simulink model "buck_circuito_completo"  (R2026a)
settings: Solver=ode23t  StopTime=12e-3  MaxStep=1e-6  RelTol=1e-4
PreLoadFcn:
  | circuito_completo_parametros;
values from neighbouring files (symbols this model uses):
  ADC_A_UV = 389000    [circuito_completo_parametros.m]
  ADC_B_X1E5 = 8251    [circuito_completo_parametros.m]
  D_FIXO_PERMIL = 500    [circuito_completo_parametros.m]
  MODO = 1    [circuito_completo.m]    (also in circuito_completo_parametros.m = 0)
  R_pot = 46.6    [circuito_completo_parametros.m]
  T_KEY = 0    [circuito_completo.m]    (also in circuito_completo_parametros.m = 0.001)
  Ts = 1e-4    (= 0.0001)    [circuito_completo_parametros.m]    (also in etapa01_referencia.m; etapa02_projeto_buck.m; etapa02_simulink.m; etapa03_projeto_ccs.m)
libraries: fl_lib x69, nesl_utility x15, ee_lib x10, simulink x1
(part 1 of 2)
settings Model: Creator=pedro  LastModifiedBy=pedro

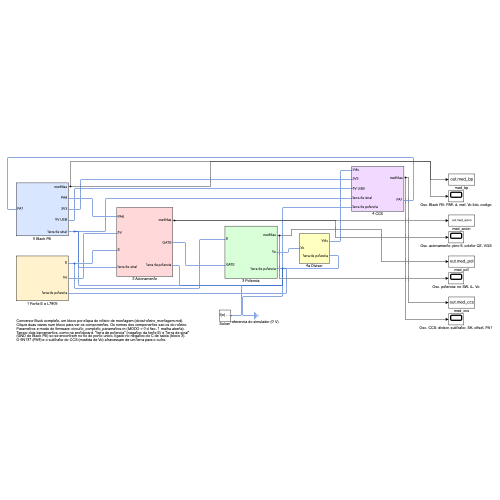
[thumbnail: Simulink's stored preview of the top-level diagram]
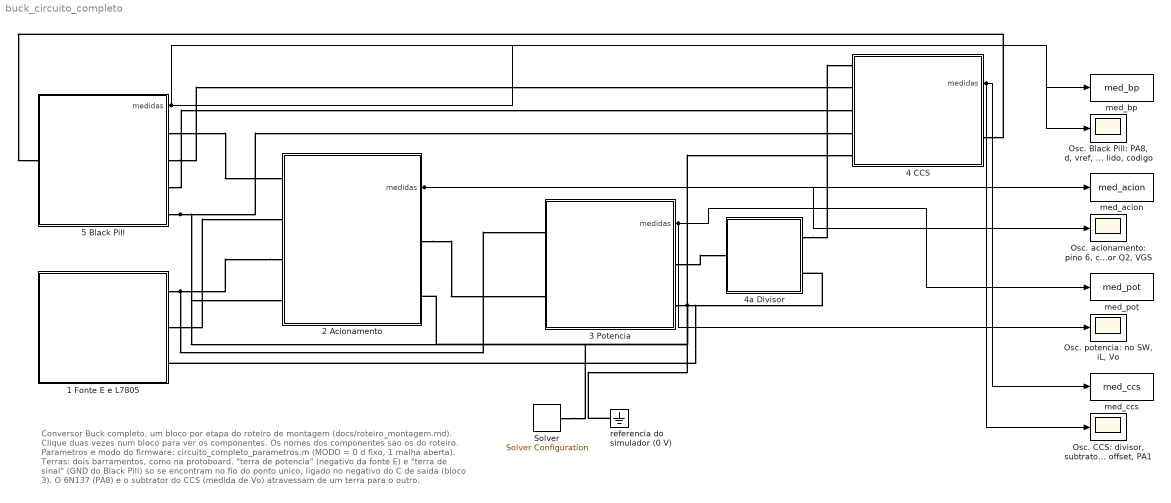
== system buck_circuito_completo ==
  note: Conversor Buck completo, um bloco por etapa do roteiro de montagem (docs/roteiro_montagem.md).
      | Clique duas vezes num bloco para ver os componentes. Os nomes dos componentes sao os do roteiro.
      | Parametros e modo do firmware: circuito_completo_parametros.m (MODO = 0 d fixo, 1 malha aberta).
      | Terras: dois barramentos, como na protoboard. "terra de potencia" (negativo da fonte E) e "terra de sinal"
      | (GND do Black Pill) so se encontram no fio do ponto unico, ligado no negativo do C de saida (bloco 3).
      | O 6N137 (PA8) e o subtrator do CCS (medida de Vo) atravessam de um terra para o outro.
  1 Fonte E e L7805 : Subsystem
  2 Acionamento : Subsystem
  3 Potencia : Subsystem
  4 CCS : Subsystem
  4a Divisor : Subsystem
  5 Black Pill : Subsystem
  "Osc. Black Pill: PA8, d, vref, Vo lido, codigo" : Scope
  "Osc. CCS: divisor, subtrator, SK, offset, PA1" : Scope
  "Osc. acionamento: pino 6, coletor Q2, VGS" : Scope
  "Osc. potencia: no SW, iL, Vo" : Scope
  Solver : nesl_utility/Solver Configuration  PhysicalDomain=network_engine_domain  SubClassName=solver  LeftPortType=input  RightPortType=generic  Tones=[]  Harmonics=[]  SimulateNoise=off  Profile=off  UseLocalSampling=off  EnableSwitchedLinearOptims=on  FrequencyDomain=off  UseCCode=off  RelTol=0.001  AbsTol=0.001  MinStep=1e-09  ToWorkspace=off  RevertToSquareIcSolve=off  NumHomotopyIterations=100  PhasorMode=off  PhasorModeNumHarmonics=1  ConsistencySolver=NEWTON_XTOL_AFTER_FTOL  CanonicalOrdering=CANONICAL  OptimizeIntermediates=OPTIMIZED  IndexReductionMethod=DerivativeReplacement  DoDC=off  ResidualTolerance=1e-09  ConsistencyTolSource=GLOBAL  ConsistencyAbsTol=0.001  ConsistencyRelTol=0.001  ConsistencyTolFactor=0.001  UseLocalSolver=off  LocalSolverChoice=NE_BACKWARD_EULER_ADVANCER  ResolveIndetEquations=on  FunctionEvalNumThread=1  LocalSolverSampleTime=0.001  DoFixedCost=off  MaxNonlinIter=3  MaxModeIter=2  ComputeImpulses=off  ImpulseIterations=2  LinearAlgebra=auto  LinearAlgebraNumThread=0  EquationFormulation=NE_TIME_EF  DelaysMemoryBudget=1024  AutomaticFiltering=on  FilteringTimeConstant=0.001  PartitionStorageMethod=AS_NEEDED  PartitionMemoryBudget=1024  PartitionMethod=ROBUST  MultibodyUseLocalSolver=off  MultibodyLocalSolverChoice=ODE1  MultibodyLocalSolverSampleTime=0.001
  med_acion : ToWorkspace  VariableName=med_acion  SaveFormat=Timeseries  SampleTime=-1
  med_bp : ToWorkspace  VariableName=med_bp  SaveFormat=Timeseries  SampleTime=-1
  med_ccs : ToWorkspace  VariableName=med_ccs  SaveFormat=Timeseries  SampleTime=-1
  med_pot : ToWorkspace  VariableName=med_pot  SaveFormat=Timeseries  SampleTime=-1
  referencia do simulador (0 V) : fl_lib/Electrical/Electrical Elements/Electrical Reference
  wires:
  5 Black Pill/1(medidas) -> med_bp/1, "Osc. Black Pill: PA8, d, vref, Vo lido, codigo"/1
  2 Acionamento/1(medidas) -> med_acion/1, "Osc. acionamento: pino 6, coletor Q2, VGS"/1
  3 Potencia/1(medidas) -> med_pot/1, "Osc. potencia: no SW, iL, Vo"/1
  4 CCS/1(medidas) -> med_ccs/1, "Osc. CCS: divisor, subtrator, SK, offset, PA1"/1
  connections:
  2 Acionamento/LConn3 -- 1 Fonte E e L7805/RConn1 -- 3 Potencia/LConn1
  1 Fonte E e L7805/RConn2 -- 2 Acionamento/LConn2
  5 Black Pill/RConn1 -- 2 Acionamento/LConn1
  2 Acionamento/RConn1 -- 3 Potencia/LConn2
  3 Potencia/RConn1 -- 4a Divisor/LConn1
  4a Divisor/RConn1 -- 4 CCS/LConn1
  5 Black Pill/RConn2 -- 4 CCS/LConn2
  5 Black Pill/RConn3 -- 4 CCS/LConn3
  4 CCS/RConn1 -- 5 Black Pill/LConn1
  1 Fonte E e L7805/RConn3 -- 3 Potencia/RConn2 -- 2 Acionamento/RConn2 -- 4a Divisor/RConn2 -- 4 CCS/LConn5 -- 5 Black Pill/RConn4 -- 2 Acionamento/LConn4 -- 4 CCS/LConn4 -- referencia do simulador (0 V)/LConn1 -- Solver/RConn1

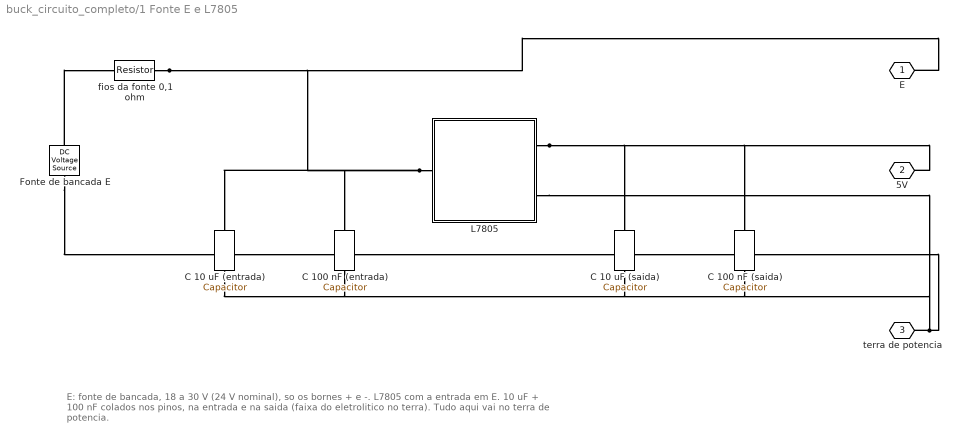
== system buck_circuito_completo/1 Fonte E e L7805 ==
  note: E: fonte de bancada, 18 a 30 V (24 V nominal), so os bornes + e -.
      | L7805 com a entrada em E. 10 uF + 100 nF colados nos pinos, na entrada e na saida (faixa do eletrolitico no terra).
      | Tudo aqui vai no terra de potencia.
  C 10 uF (entrada) : fl_lib/Electrical/Electrical Elements/Capacitor  c=10e-6 F  r=0.3 Ohm  g=0 1/Ohm  i_specify=off  i_priority=None  i=0 A  i_nominal_specify=off  i_nominal_value=1  i_nominal_unit=A  v_specify=off  v_priority=None  v=0 V  v_nominal_specify=off  v_nominal_value=1  v_nominal_unit=V  vc_specify=off  vc_priority=High  vc=0 V  vc_nominal_specify=off  vc_nominal_value=1  vc_nominal_unit=V
  C 10 uF (saida) : fl_lib/Electrical/Electrical Elements/Capacitor  c=10e-6 F  r=0.3 Ohm  g=0 1/Ohm  i_specify=off  i_priority=None  i=0 A  i_nominal_specify=off  i_nominal_value=1  i_nominal_unit=A  v_specify=off  v_priority=None  v=0 V  v_nominal_specify=off  v_nominal_value=1  v_nominal_unit=V  vc_specify=off  vc_priority=High  vc=0 V  vc_nominal_specify=off  vc_nominal_value=1  vc_nominal_unit=V
  C 100 nF (entrada) : fl_lib/Electrical/Electrical Elements/Capacitor  c=100e-9 F  r=1e-6 Ohm  g=0 1/Ohm  i_specify=off  i_priority=None  i=0 A  i_nominal_specify=off  i_nominal_value=1  i_nominal_unit=A  v_specify=off  v_priority=None  v=0 V  v_nominal_specify=off  v_nominal_value=1  v_nominal_unit=V  vc_specify=off  vc_priority=High  vc=0 V  vc_nominal_specify=off  vc_nominal_value=1  vc_nominal_unit=V
  C 100 nF (saida) : fl_lib/Electrical/Electrical Elements/Capacitor  c=100e-9 F  r=1e-6 Ohm  g=0 1/Ohm  i_specify=off  i_priority=None  i=0 A  i_nominal_specify=off  i_nominal_value=1  i_nominal_unit=A  v_specify=off  v_priority=None  v=0 V  v_nominal_specify=off  v_nominal_value=1  v_nominal_unit=V  vc_specify=off  vc_priority=High  vc=0 V  vc_nominal_specify=off  vc_nominal_value=1  vc_nominal_unit=V
  Fonte de bancada E : fl_lib/Electrical/Electrical Sources/DC Voltage Source  v0=E V
  L7805 : Subsystem
  fios da fonte 0,1 ohm : fl_lib/Electrical/Electrical Elements/Resistor  R=0.1 Ohm  i_specify=off  i_priority=None  i=0 A  i_nominal_specify=off  i_nominal_value=1  i_nominal_unit=A  v_specify=off  v_priority=None  v=0 V  v_nominal_specify=off  v_nominal_value=1  v_nominal_unit=V
  E : PMIOPort  Side=Right
  5V : PMIOPort  Port=2  Side=Right
  terra de potencia : PMIOPort  Port=3  Side=Right
  connections:
  Fonte de bancada E/LConn1 -- fios da fonte 0,1 ohm/LConn1
  E/RConn1 -- fios da fonte 0,1 ohm/RConn1 -- C 10 uF (entrada)/LConn1 -- L7805/LConn1 -- C 100 nF (entrada)/LConn1
  Fonte de bancada E/RConn1 -- L7805/RConn2 -- C 10 uF (entrada)/RConn1 -- C 100 nF (entrada)/RConn1 -- C 10 uF (saida)/RConn1 -- terra de potencia/RConn1 -- C 100 nF (saida)/RConn1
  5V/RConn1 -- L7805/RConn1 -- C 10 uF (saida)/LConn1 -- C 100 nF (saida)/LConn1

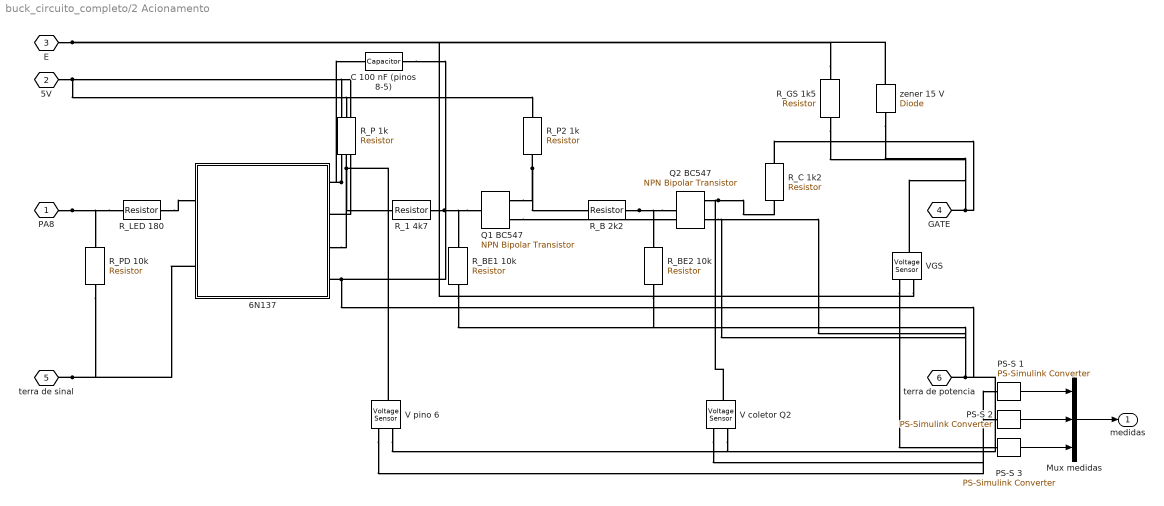
== system buck_circuito_completo/2 Acionamento ==
  6N137 : Subsystem
  C 100 nF (pinos 8-5) : fl_lib/Electrical/Electrical Elements/Capacitor  c=100e-9 F  r=1e-6 Ohm  g=0 1/Ohm  i_specify=off  i_priority=None  i=0 A  i_nominal_specify=off  i_nominal_value=1  i_nominal_unit=A  v_specify=off  v_priority=None  v=0 V  v_nominal_specify=off  v_nominal_value=1  v_nominal_unit=V  vc_specify=off  vc_priority=High  vc=0 V  vc_nominal_specify=off  vc_nominal_value=1  vc_nominal_unit=V
  Mux medidas : Mux  Inputs=3
  PS-S 1 : nesl_utility/PS-Simulink Converter  PhysicalDomain=network_engine_domain  SubClassName=ps_output  LeftPortType=input  RightPortType=output  PseudoPeriodic=off  Frequencies=[]  VectorFormat=inherit  Unit=V  AffineConversion=off
  PS-S 2 : nesl_utility/PS-Simulink Converter  PhysicalDomain=network_engine_domain  SubClassName=ps_output  LeftPortType=input  RightPortType=output  PseudoPeriodic=off  Frequencies=[]  VectorFormat=inherit  Unit=V  AffineConversion=off
  PS-S 3 : nesl_utility/PS-Simulink Converter  PhysicalDomain=network_engine_domain  SubClassName=ps_output  LeftPortType=input  RightPortType=output  PseudoPeriodic=off  Frequencies=[]  VectorFormat=inherit  Unit=V  AffineConversion=off
  Q1 BC547 : ee_lib/Semiconductors & Converters/NPN Bipolar Transistor  parameterization=1  BF=100  IS=1e-14 A  VAF=200 V  hfe=100  hoe=50e-6 1/Ohm  Ic_h=1 mA  Vce_h=5 V  V1=0.55 V  I1=0.5 mA  BR=1  Tmeas=25 degC  RC=0.01 Ohm  RE=1e-4 Ohm  RB=1 Ohm  C_BC=5 pF  C_BE=5 pF  TF=0 us  TR=0 us  prmDatasheet=1  prmEquCoeff=1  hfe_T2=125  XTB=0  V1_T2=0.45 V  I1_T2=0.5 mA  Tmeas2=125 degC  EG=1.11 eV  XTI=3  TdeviceDatasheet=25 degC  TdeviceEquCoeff=25 degC  ec=1  ib_specify=off  ib_priority=None  ib=0 A  ib_nominal_specify=off  ib_nominal_value=1  ib_nominal_unit=A  ic_specify=off  ic_priority=None  ic=0 A  ic_nominal_specify=off  ic_nominal_value=1  ic_nominal_unit=A  vce_specify=off  vce_priority=None  vce=0 V  vce_nominal_specify=off  vce_nominal_value=1  vce_nominal_unit=V  vbe_specify=off  vbe_priority=None  vbe=0 V  vbe_nominal_specify=off  vbe_nominal_value=1  vbe_nominal_unit=V  Qbc_specify=off  Qbc_priority=High  Qbc=0 C  Qbc_nominal_specify=off  Qbc_nominal_value=1  Qbc_nominal_unit=uC  Qbe_specify=off  Qbe_priority=High  Qbe=0 C  Qbe_nominal_specify=off  Qbe_nominal_value=1  Qbe_nominal_unit=uC  thermal_network_parameterization=ee.enum.thermalNetworkTopology.junctionCase  Rth=[0, 10] K/W  Rth_Cauer=[1, 3, 10] K/W  Rth_Foster=[.08, .14, .22, .16] K/W  thermal_mass_parameterization=ee.enum.thermalNetwork.timeconstant  thermal_mass=[0, 1] J/K  thermal_mass_Cauer=[.1, .3, 1] J/K  thermal_mass_Foster=[.001, .005, .05, .5] J/K  thermal_time_constant=[0, 10] s  thermal_time_constant_Cauer=[1, 3, 10] s  thermal_time_constant_Foster=[7e-05, .0007, .01, .08] s  thermal_mass_initial_temperatures=[25, 25] degC  thermal_mass_initial_temperatures_Cauer=[25, 25, 25] degC  Tvec_initial_Foster=[25, 25, 25, 25] degC
  Q2 BC547 : ee_lib/Semiconductors & Converters/NPN Bipolar Transistor  parameterization=1  BF=100  IS=1e-14 A  VAF=200 V  hfe=100  hoe=50e-6 1/Ohm  Ic_h=1 mA  Vce_h=5 V  V1=0.55 V  I1=0.5 mA  BR=1  Tmeas=25 degC  RC=0.01 Ohm  RE=1e-4 Ohm  RB=1 Ohm  C_BC=5 pF  C_BE=5 pF  TF=0 us  TR=0 us  prmDatasheet=1  prmEquCoeff=1  hfe_T2=125  XTB=0  V1_T2=0.45 V  I1_T2=0.5 mA  Tmeas2=125 degC  EG=1.11 eV  XTI=3  TdeviceDatasheet=25 degC  TdeviceEquCoeff=25 degC  ec=1  ib_specify=off  ib_priority=None  ib=0 A  ib_nominal_specify=off  ib_nominal_value=1  ib_nominal_unit=A  ic_specify=off  ic_priority=None  ic=0 A  ic_nominal_specify=off  ic_nominal_value=1  ic_nominal_unit=A  vce_specify=off  vce_priority=None  vce=0 V  vce_nominal_specify=off  vce_nominal_value=1  vce_nominal_unit=V  vbe_specify=off  vbe_priority=None  vbe=0 V  vbe_nominal_specify=off  vbe_nominal_value=1  vbe_nominal_unit=V  Qbc_specify=off  Qbc_priority=High  Qbc=0 C  Qbc_nominal_specify=off  Qbc_nominal_value=1  Qbc_nominal_unit=uC  Qbe_specify=off  Qbe_priority=High  Qbe=0 C  Qbe_nominal_specify=off  Qbe_nominal_value=1  Qbe_nominal_unit=uC  thermal_network_parameterization=ee.enum.thermalNetworkTopology.junctionCase  Rth=[0, 10] K/W  Rth_Cauer=[1, 3, 10] K/W  Rth_Foster=[.08, .14, .22, .16] K/W  thermal_mass_parameterization=ee.enum.thermalNetwork.timeconstant  thermal_mass=[0, 1] J/K  thermal_mass_Cauer=[.1, .3, 1] J/K  thermal_mass_Foster=[.001, .005, .05, .5] J/K  thermal_time_constant=[0, 10] s  thermal_time_constant_Cauer=[1, 3, 10] s  thermal_time_constant_Foster=[7e-05, .0007, .01, .08] s  thermal_mass_initial_temperatures=[25, 25] degC  thermal_mass_initial_temperatures_Cauer=[25, 25, 25] degC  Tvec_initial_Foster=[25, 25, 25, 25] degC
  R_1 4k7 : fl_lib/Electrical/Electrical Elements/Resistor  R=4.7e3 Ohm  i_specify=off  i_priority=None  i=0 A  i_nominal_specify=off  i_nominal_value=1  i_nominal_unit=A  v_specify=off  v_priority=None  v=0 V  v_nominal_specify=off  v_nominal_value=1  v_nominal_unit=V
  R_B 2k2 : fl_lib/Electrical/Electrical Elements/Resistor  R=2.2e3 Ohm  i_specify=off  i_priority=None  i=0 A  i_nominal_specify=off  i_nominal_value=1  i_nominal_unit=A  v_specify=off  v_priority=None  v=0 V  v_nominal_specify=off  v_nominal_value=1  v_nominal_unit=V
  R_BE1 10k : fl_lib/Electrical/Electrical Elements/Resistor  R=10e3 Ohm  i_specify=off  i_priority=None  i=0 A  i_nominal_specify=off  i_nominal_value=1  i_nominal_unit=A  v_specify=off  v_priority=None  v=0 V  v_nominal_specify=off  v_nominal_value=1  v_nominal_unit=V
  R_BE2 10k : fl_lib/Electrical/Electrical Elements/Resistor  R=10e3 Ohm  i_specify=off  i_priority=None  i=0 A  i_nominal_specify=off  i_nominal_value=1  i_nominal_unit=A  v_specify=off  v_priority=None  v=0 V  v_nominal_specify=off  v_nominal_value=1  v_nominal_unit=V
  R_C 1k2 : fl_lib/Electrical/Electrical Elements/Resistor  R=1.2e3 Ohm  i_specify=off  i_priority=None  i=0 A  i_nominal_specify=off  i_nominal_value=1  i_nominal_unit=A  v_specify=off  v_priority=None  v=0 V  v_nominal_specify=off  v_nominal_value=1  v_nominal_unit=V
  R_GS 1k5 : fl_lib/Electrical/Electrical Elements/Resistor  R=1.5e3 Ohm  i_specify=off  i_priority=None  i=0 A  i_nominal_specify=off  i_nominal_value=1  i_nominal_unit=A  v_specify=off  v_priority=None  v=0 V  v_nominal_specify=off  v_nominal_value=1  v_nominal_unit=V
  R_LED 180 : fl_lib/Electrical/Electrical Elements/Resistor  R=180 Ohm  i_specify=off  i_priority=None  i=0 A  i_nominal_specify=off  i_nominal_value=1  i_nominal_unit=A  v_specify=off  v_priority=None  v=0 V  v_nominal_specify=off  v_nominal_value=1  v_nominal_unit=V
  R_P 1k : fl_lib/Electrical/Electrical Elements/Resistor  R=1e3 Ohm  i_specify=off  i_priority=None  i=0 A  i_nominal_specify=off  i_nominal_value=1  i_nominal_unit=A  v_specify=off  v_priority=None  v=0 V  v_nominal_specify=off  v_nominal_value=1  v_nominal_unit=V
  R_P2 1k : fl_lib/Electrical/Electrical Elements/Resistor  R=1e3 Ohm  i_specify=off  i_priority=None  i=0 A  i_nominal_specify=off  i_nominal_value=1  i_nominal_unit=A  v_specify=off  v_priority=None  v=0 V  v_nominal_specify=off  v_nominal_value=1  v_nominal_unit=V
  R_PD 10k : fl_lib/Electrical/Electrical Elements/Resistor  R=10e3 Ohm  i_specify=off  i_priority=None  i=0 A  i_nominal_specify=off  i_nominal_value=1  i_nominal_unit=A  v_specify=off  v_priority=None  v=0 V  v_nominal_specify=off  v_nominal_value=1  v_nominal_unit=V
  V coletor Q2 : fl_lib/Electrical/Electrical Sensors/Voltage Sensor
  V pino 6 : fl_lib/Electrical/Electrical Sensors/Voltage Sensor
  VGS : fl_lib/Electrical/Electrical Sensors/Voltage Sensor
  zener 15 V : ee_lib/Semiconductors & Converters/Diode  ModelType=ee.enum.diode.modelType.pwl  TableType=ee.enum.diode.tableType.IfMat  IfMat=[.07, .12, .19, 1.75, 4.24, 7.32, 11.2; .16, .3, .72, 2.14, 5.02, 8.35, 13.12] A  VfMat=[.9, 1.15, 1.25, 1.5, 1.75, 2.17, 2.6, 2.85; .58, .68, .75, 1.1, 1.38, 1.77, 2.27, 2.7] V  TjVec=[25, 125] degC  VfVec=[.5, .7, .9, 1.3, 1.7, 2.1, 2.5] V  IfVec=[.1, .2, .5, 1, 2, 4, 7, 10] A  IrMat=[1e-06, 2e-06, 5e-06, 1e-05, 2.5e-05, 5e-05, .0001; 2e-06, 5e-06, 1e-05, 4e-05, 8e-05, .0002, .0005] A  VrMat=[10, 100, 200, 250, 300, 325, 350; 10, 70, 160, 220, 270, 300, 320] V  VrVec=[10, 20, 40, 50, 70, 80, 100] V  IrVec=[1e-06, 2e-06, 5e-06, 1e-05, 2e-05, 5e-05, .0001] A  Vf=0.7 V  Ron=0.5 Ohm  Goff=1e-8 S  prmExp=ee.enum.diode.expParam.useTwo  I12=[.0137, .545] A  V12=[.6, .7] V  RS=0 Ohm  Tmeas=298.15 K  IS=1e-12 A  ec=1  I1=0.0137 A  V1=0.6 V  N_series=1  N_parallel=1  ZenerEnable=true  Rz=1 Ohm  BV=15 V  C_param=ee.enum.diode.capParam.fixed  CJ=0 pF  CJ0=5 pF  Vvec=[.1, 10, 100] V  Cvec=[3.5, 1, .4] pF  VJ=1 V  Mgrad=0.5  FC=0.5  Q_param=ee.enum.diode.recoveryParam.off  iRM=-7.15 A  iF=4 A  didt=-750 A/us  trr_factor=3  trr=115 ns  Qrr=150 nA*s  Vr=-600 V  Ls=150 nH  Erec=0.03 J  TT=50 ns  tau=100 ns  T_param=ee.enum.diode.temperatureParam.off  Tdevice=298.15 K  I1_T2=0.245 A  V1_T2=0.5 V  IS_T2=1.25e-7 A  Tmeas2=125 degC  XTI_param=ee.enum.diode.xtiParam.pn  XTI=3  EG_param=ee.enum.diode.egapParam.material_si  EG=1.11 eV  dBVdT=0 V/K  enable_fault_input=simscape.enum.onoff.off  i_specify=off  i_priority=None  i=0 A  i_nominal_specify=off  i_nominal_value=1  i_nominal_unit=A  v_specify=off  v_priority=None  v=0 V  v_nominal_specify=off  v_nominal_value=1  v_nominal_unit=V  v_capacitor_specify=off  v_capacitor_priority=None  v_capacitor=0 V  v_capacitor_nominal_specify=off  v_capacitor_nominal_value=1  v_capacitor_nominal_unit=V  Qj_specify=off  Qj_priority=High  Qj=0 C  Qj_nominal_specify=off  Qj_nominal_value=1  Qj_nominal_unit=C  i_diode_specify=off  i_diode_priority=None  i_diode=0 A  i_diode_nominal_specify=off  i_diode_nominal_value=1  i_diode_nominal_unit=A  v_diode_specify=off  v_diode_priority=None  v_diode=0 V  v_diode_nominal_specify=off  v_diode_nominal_value=1  v_diode_nominal_unit=V  i_capacitor_specify=off  i_capacitor_priority=None  i_capacitor=0 A  i_capacitor_nominal_specify=off  i_capacitor_nominal_value=1  i_capacitor_nominal_unit=A  fidelity_level=ee.enum.diode.fidelity.includeChargeDyn  rec_loss_model=ee.enum.diode.reverseRecoveryModelTabulateUpTo3D.fixed  ErecVal=0 J  scaleWithIandV=true  ErecMat=zeros(2, 3) J  ErecMat3D=zeros(2, 3, 2) J  TjrecVec=[298.15, 398.15] K  IfrecVec=[.1, 1, 10] A  IrecVal=10 A  VrecVal=10 V  VrecVec=[0, 100] V  tFilter=1 / 1000 / 100 s  thermal_network_parameterization=ee.enum.thermalNetworkTopology.junctionCase  Rth=[0, 10] K/W  Rth_Cauer=[1, 3, 10] K/W  Rth_Foster=[.08, .14, .22, .16] K/W  thermal_mass_parameterization=ee.enum.thermalNetwork.timeconstant  thermal_mass=[0, 1] J/K  thermal_mass_Cauer=[.1, .3, 1] J/K  thermal_mass_Foster=[.001, .005, .05, .5] J/K  thermal_time_constant=[0, 10] s  thermal_time_constant_Cauer=[1, 3, 10] s  thermal_time_constant_Foster=[7e-05, .0007, .01, .08] s  thermal_mass_initial_temperatures=[25, 25] degC  thermal_mass_initial_temperatures_Cauer=[25, 25, 25] degC  junction_thermal_mass=0.01 J/K  Tvec_initial_Foster=[25, 25, 25, 25] degC  no_thermal_network=0  junction_temperature_specify=off  junction_temperature_priority=None  junction_temperature=25 degC  junction_temperature_nominal_specify=off  junction_temperature_nominal_value=1  junction_temperature_nominal_unit=degC
  PA8 : PMIOPort  Side=Left
  5V : PMIOPort  Port=2  Side=Left
  E : PMIOPort  Port=3  Side=Left
  GATE : PMIOPort  Port=4  Side=Right
  terra de sinal : PMIOPort  Port=5  Side=Left
  terra de potencia : PMIOPort  Port=6  Side=Right
  medidas : Outport
  wires:
  Mux medidas/1 -> medidas/1
  PS-S 1/1 -> Mux medidas/1
  PS-S 2/1 -> Mux medidas/2
  PS-S 3/1 -> Mux medidas/3
  connections:
  R_LED 180/LConn1 -- PA8/RConn1 -- R_PD 10k/LConn1
  terra de sinal/RConn1 -- R_PD 10k/RConn1 -- 6N137/LConn2
  R_LED 180/RConn1 -- 6N137/LConn1
  5V/RConn1 -- 6N137/RConn2 -- 6N137/RConn1 -- C 100 nF (pinos 8-5)/LConn1 -- R_P 1k/LConn1 -- R_P2 1k/LConn1
  6N137/RConn4 -- C 100 nF (pinos 8-5)/RConn1 -- R_BE1 10k/RConn1 -- Q1 BC547/RConn2 -- R_BE2 10k/RConn1 -- Q2 BC547/RConn2 -- V pino 6/RConn2 -- terra de potencia/RConn1 -- V coletor Q2/RConn2
  6N137/RConn3 -- R_1 4k7/LConn1 -- R_P 1k/RConn1 -- V pino 6/LConn1
  Q1 BC547/LConn1 -- R_1 4k7/RConn1 -- R_BE1 10k/LConn1
  R_P2 1k/RConn1 -- Q1 BC547/RConn1 -- R_B 2k2/LConn1
  Q2 BC547/LConn1 -- R_B 2k2/RConn1 -- R_BE2 10k/LConn1
  R_C 1k2/RConn1 -- Q2 BC547/RConn1 -- V coletor Q2/LConn1
  R_C 1k2/LConn1 -- R_GS 1k5/RConn1 -- zener 15 V/LConn1 -- GATE/RConn1 -- VGS/LConn1
  R_GS 1k5/LConn1 -- E/RConn1 -- zener 15 V/RConn1 -- VGS/RConn2
  V pino 6/RConn1 -- PS-S 1/LConn1
  V coletor Q2/RConn1 -- PS-S 2/LConn1
  VGS/RConn1 -- PS-S 3/LConn1

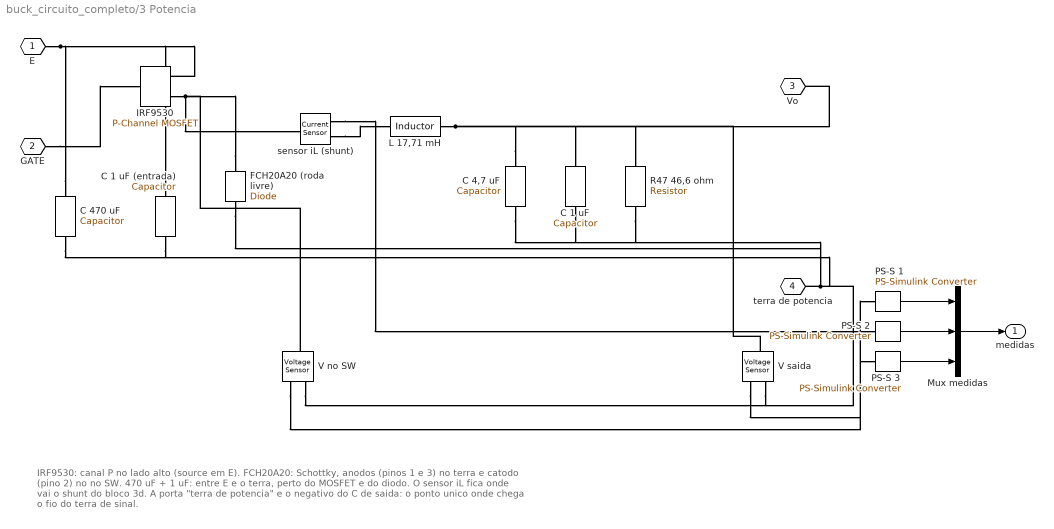
== system buck_circuito_completo/3 Potencia ==
  note: IRF9530: canal P no lado alto (source em E). FCH20A20: Schottky, anodos (pinos 1 e 3) no terra e catodo (pino 2) no no SW.
      | 470 uF + 1 uF: entre E e o terra, perto do MOSFET e do diodo. O sensor iL fica onde vai o shunt do bloco 3d.
      | A porta "terra de potencia" e o negativo do C de saida: o ponto unico onde chega o fio do terra de sinal.
  C 1 uF : fl_lib/Electrical/Electrical Elements/Capacitor  c=C_out2 F  r=1e-6 Ohm  g=0 1/Ohm  i_specify=off  i_priority=None  i=0 A  i_nominal_specify=off  i_nominal_value=1  i_nominal_unit=A  v_specify=off  v_priority=None  v=0 V  v_nominal_specify=off  v_nominal_value=1  v_nominal_unit=V  vc_specify=off  vc_priority=High  vc=0 V  vc_nominal_specify=off  vc_nominal_value=1  vc_nominal_unit=V
  C 1 uF (entrada) : fl_lib/Electrical/Electrical Elements/Capacitor  c=1e-6 F  r=1e-6 Ohm  g=0 1/Ohm  i_specify=off  i_priority=None  i=0 A  i_nominal_specify=off  i_nominal_value=1  i_nominal_unit=A  v_specify=off  v_priority=None  v=0 V  v_nominal_specify=off  v_nominal_value=1  v_nominal_unit=V  vc_specify=off  vc_priority=High  vc=0 V  vc_nominal_specify=off  vc_nominal_value=1  vc_nominal_unit=V
  C 4,7 uF : fl_lib/Electrical/Electrical Elements/Capacitor  c=C_out1 F  r=1e-6 Ohm  g=0 1/Ohm  i_specify=off  i_priority=None  i=0 A  i_nominal_specify=off  i_nominal_value=1  i_nominal_unit=A  v_specify=off  v_priority=None  v=0 V  v_nominal_specify=off  v_nominal_value=1  v_nominal_unit=V  vc_specify=off  vc_priority=High  vc=0 V  vc_nominal_specify=off  vc_nominal_value=1  vc_nominal_unit=V
  C 470 uF : fl_lib/Electrical/Electrical Elements/Capacitor  c=470e-6 F  r=0.1 Ohm  g=0 1/Ohm  i_specify=off  i_priority=None  i=0 A  i_nominal_specify=off  i_nominal_value=1  i_nominal_unit=A  v_specify=off  v_priority=None  v=0 V  v_nominal_specify=off  v_nominal_value=1  v_nominal_unit=V  vc_specify=off  vc_priority=High  vc=0 V  vc_nominal_specify=off  vc_nominal_value=1  vc_nominal_unit=V
  FCH20A20 (roda livre) : ee_lib/Semiconductors & Converters/Diode  ModelType=ee.enum.diode.modelType.pwl  TableType=ee.enum.diode.tableType.IfMat  IfMat=[.07, .12, .19, 1.75, 4.24, 7.32, 11.2; .16, .3, .72, 2.14, 5.02, 8.35, 13.12] A  VfMat=[.9, 1.15, 1.25, 1.5, 1.75, 2.17, 2.6, 2.85; .58, .68, .75, 1.1, 1.38, 1.77, 2.27, 2.7] V  TjVec=[25, 125] degC  VfVec=[.5, .7, .9, 1.3, 1.7, 2.1, 2.5] V  IfVec=[.1, .2, .5, 1, 2, 4, 7, 10] A  IrMat=[1e-06, 2e-06, 5e-06, 1e-05, 2.5e-05, 5e-05, .0001; 2e-06, 5e-06, 1e-05, 4e-05, 8e-05, .0002, .0005] A  VrMat=[10, 100, 200, 250, 300, 325, 350; 10, 70, 160, 220, 270, 300, 320] V  VrVec=[10, 20, 40, 50, 70, 80, 100] V  IrVec=[1e-06, 2e-06, 5e-06, 1e-05, 2e-05, 5e-05, .0001] A  Vf=0.55 V  Ron=0.03 Ohm  Goff=1e-8 S  prmExp=ee.enum.diode.expParam.useTwo  I12=[.0137, .545] A  V12=[.6, .7] V  RS=0 Ohm  Tmeas=298.15 K  IS=1e-12 A  ec=1  I1=0.0137 A  V1=0.6 V  N_series=1  N_parallel=1  ZenerEnable=false  Rz=0.3 Ohm  BV=30 V  C_param=ee.enum.diode.capParam.fixed  CJ=0 pF  CJ0=5 pF  Vvec=[.1, 10, 100] V  Cvec=[3.5, 1, .4] pF  VJ=1 V  Mgrad=0.5  FC=0.5  Q_param=ee.enum.diode.recoveryParam.off  iRM=-7.15 A  iF=4 A  didt=-750 A/us  trr_factor=3  trr=115 ns  Qrr=150 nA*s  Vr=-600 V  Ls=150 nH  Erec=0.03 J  TT=50 ns  tau=100 ns  T_param=ee.enum.diode.temperatureParam.off  Tdevice=298.15 K  I1_T2=0.245 A  V1_T2=0.5 V  IS_T2=1.25e-7 A  Tmeas2=125 degC  XTI_param=ee.enum.diode.xtiParam.pn  XTI=3  EG_param=ee.enum.diode.egapParam.material_si  EG=1.11 eV  dBVdT=0 V/K  enable_fault_input=simscape.enum.onoff.off  i_specify=off  i_priority=None  i=0 A  i_nominal_specify=off  i_nominal_value=1  i_nominal_unit=A  v_specify=off  v_priority=None  v=0 V  v_nominal_specify=off  v_nominal_value=1  v_nominal_unit=V  v_capacitor_specify=off  v_capacitor_priority=None  v_capacitor=0 V  v_capacitor_nominal_specify=off  v_capacitor_nominal_value=1  v_capacitor_nominal_unit=V  Qj_specify=off  Qj_priority=High  Qj=0 C  Qj_nominal_specify=off  Qj_nominal_value=1  Qj_nominal_unit=C  i_diode_specify=off  i_diode_priority=None  i_diode=0 A  i_diode_nominal_specify=off  i_diode_nominal_value=1  i_diode_nominal_unit=A  v_diode_specify=off  v_diode_priority=None  v_diode=0 V  v_diode_nominal_specify=off  v_diode_nominal_value=1  v_diode_nominal_unit=V  i_capacitor_specify=off  i_capacitor_priority=None  i_capacitor=0 A  i_capacitor_nominal_specify=off  i_capacitor_nominal_value=1  i_capacitor_nominal_unit=A  fidelity_level=ee.enum.diode.fidelity.includeChargeDyn  rec_loss_model=ee.enum.diode.reverseRecoveryModelTabulateUpTo3D.fixed  ErecVal=0 J  scaleWithIandV=true  ErecMat=zeros(2, 3) J  ErecMat3D=zeros(2, 3, 2) J  TjrecVec=[298.15, 398.15] K  IfrecVec=[.1, 1, 10] A  IrecVal=10 A  VrecVal=10 V  VrecVec=[0, 100] V  tFilter=1 / 1000 / 100 s  thermal_network_parameterization=ee.enum.thermalNetworkTopology.junctionCase  Rth=[0, 10] K/W  Rth_Cauer=[1, 3, 10] K/W  Rth_Foster=[.08, .14, .22, .16] K/W  thermal_mass_parameterization=ee.enum.thermalNetwork.timeconstant  thermal_mass=[0, 1] J/K  thermal_mass_Cauer=[.1, .3, 1] J/K  thermal_mass_Foster=[.001, .005, .05, .5] J/K  thermal_time_constant=[0, 10] s  thermal_time_constant_Cauer=[1, 3, 10] s  thermal_time_constant_Foster=[7e-05, .0007, .01, .08] s  thermal_mass_initial_temperatures=[25, 25] degC  thermal_mass_initial_temperatures_Cauer=[25, 25, 25] degC  junction_thermal_mass=0.01 J/K  Tvec_initial_Foster=[25, 25, 25, 25] degC  no_thermal_network=0  junction_temperature_specify=off  junction_temperature_priority=None  junction_temperature=25 degC  junction_temperature_nominal_specify=off  junction_temperature_nominal_value=1  junction_temperature_nominal_unit=degC
  IRF9530 : ee_lib/Semiconductors & Converters/P-Channel MOSFET  paramTerminal=ee.enum.mosfet.numberOfTerminals.three  parameterization=ee.enum.mosfet.parameterization.datasheet  Beta=2.0 A/V^2  Rds=0.3 Ohm  Id=-7 A  Vgs=-10 V  Vth=-3 V  Vth0=-1.4 V  lam=0 1/V  gamma_vth=0.5 V^(1/2)  phib=0.5 V  Vth1=-1.6071 V  Vbs1=1 V  Vth2=-1.7660 V  Vbs2=2 V  Tmeas=25 degC  Vsg_vec=[-1, -.5, 2, 3, 4, 5] V  Vsd_vec=[0, 2, 4, 8, 12, 16, 20] V  Vsb_vec=[0, -4, -6, -12] V  T_vec=[25, 125] degC  Vth_vec=[-.4, -1.2, -1.4, -1.45] V  Vth_mat=[-.4, -.35; -1.2, -1.15; -1.4, -1.35; -1.45, -1.4] V  Isd_mat=[0, 0, 0, 0, 0, 0, 0; 0, 0, 0, 0, 0, 0, 0; 0, .003, .0038, .0043, .0046, .0048, .0049; 0, .0055, .008, .009, .0095, .01, .0101; 0, .0115, .016, .018, .019, .0195, .02; 0, .0152, .0225, .0265, .028, .0295, .03] A  Isd_mat0=[0, 0, 0, 0, 0, 0, 0; 0, 0, 0, 0, 0, 0, 0; 0, .003, .0038, .0043, .0046, .0048, .0049; 0, .0055, .008, .009, .0095, .01, .0101; 0, .0115, .016, .018, .019, .0195, .02; 0, .0152, .0225, .0265, .028, .0295, .03] A  Isd_mat_3D=zeros(6, 7, 2) A  Isd_mat_3D0=zeros(6, 7, 2) A  IV_table_symmetry=ee.enum.mosfet.symmetricPIV.no  RS=0.0001 Ohm  RD=0.01 Ohm  RB=0.001 Ohm  LeadRs=0 Ohm  LeadRd=0 Ohm  LeadRg=0 Ohm  LeadRb=0 Ohm  LS=0 nH  LD=0 nH  LG=0 nH  LB=0 nH  C_param=ee.enum.mosfet.capacitanceParam.fixedciss  C_GS=158 pF  C_GD=24 pF  C_GB=0 pF  C_DS=0 pF  C_iss=760 pF  C_rss=140 pF  C_oss=0 pF  C_iss_vec=[225, 210, 200, 185, 175, 170] pF  C_rss_vec=[75, 60, 50, 35, 25, 20] pF  C_oss_vec=[180, 160, 125, 80, 60, 45] pF  C_GS_vec=[150, 150, 150, 150, 150, 150] pF  C_GD_vec=[75, 60, 50, 35, 25, 20] pF  C_GB_vec=[450, 400, 300, 190, 95, 55] pF  C_Vsg_vec=0 V  C_DS_vec=[105, 100, 75, 45, 35, 25] pF  C_Vsd_vec=[.1, .3, 1, 3, 10, 30] V  V_GS_for_cap_data=0 V  charge_linearity_param=ee.enum.mosfet.cgdLinearity.constant  C_OX=200 pF  V_C_OX=0.5 V  charge_linearity_param_vgb=ee.enum.mosfet.cgbLinearity.instantly  charge_linearity_param_with_vgb=ee.enum.mosfet.cgbLinearityWithSeparateCgb.instantly  Di_param=ee.enum.mosfet.diodeParam.no  IsDiode=1e-12 A  Vbi=0.6 V  n=1  Cj0Diode=0 pF  TT=50e-9 s  Tmeas_dio=25 degC  TableTypeNoT=ee.enum.mosfet.tableType.IfMat  TableType=ee.enum.diode.tableType.IfMat  IfVec=[.07, .12, .19, 1.75, 4.24, 7.32, 11.2] A  IfMat=[.07, .12, .19, 1.75, 4.24, 7.32, 11.2; .16, .3, .72, 2.14, 4.02, 6.35, 9.12] A  VfVecV=[.9, 1.15, 1.25, 1.5, 1.75, 2.17, 2.6, 2.85] V  VfMatV=[.9, 1.15, 1.25, 1.5, 1.75, 2.17, 2.6, 2.85; .58, .68, .75, 1.1, 1.38, 1.77, 2.27, 2.7] V  TjVec=[25, 125] degC  VfVec=[.5, .7, .9, 1.3, 1.7, 2.1, 2.5] V  IfVecV=[.1, .2, .5, 1, 2, 4, 7, 10] A  diode_Goff=1e-12 1/Ohm  prmDatasheet=ee.enum.temperatureParameterization.none  prmEquCoeff=ee.enum.temperatureParameterization.none  dVth_dT=2 mV/K  dVth0_dT=2 mV/K  Rds_T2=0.25 Ohm  BEXDatasheet=-1.5  BEXEquCoeff=-1.5  etaisDatasheet=3  etaisEquCoeff=3  Tmeas2=125 degC  etaisTabulated=3  TdeviceDatasheet=25 degC  TdeviceEquCoeff=25 degC  TdeviceTabulated=25 degC  i_g_specify=off  i_g_priority=None  i_g=0 A  i_g_nominal_specify=off  i_g_nominal_value=1  i_g_nominal_unit=A  i_d_specify=off  i_d_priority=None  i_d=0 A  i_d_nominal_specify=off  i_d_nominal_value=1  i_d_nominal_unit=A  i_b_specify=off  i_b_priority=None  i_b=0 A  i_b_nominal_specify=off  i_b_nominal_value=1  i_b_nominal_unit=A  voltage_gs_specify=off  voltage_gs_priority=None  voltage_gs=0 V  voltage_gs_nominal_specify=off  voltage_gs_nominal_value=1  voltage_gs_nominal_unit=V  voltage_ds_specify=off  voltage_ds_priority=None  voltage_ds=0 V  voltage_ds_nominal_specify=off  voltage_ds_nominal_value=1  voltage_ds_nominal_unit=V  voltage_bs_specify=off  voltage_bs_priority=None  voltage_bs=0 V  voltage_bs_nominal_specify=off  voltage_bs_nominal_value=1  voltage_bs_nominal_unit=V  v_Cgs_specify=off  v_Cgs_priority=High  v_Cgs=0 V  v_Cgs_nominal_specify=off  v_Cgs_nominal_value=1  v_Cgs_nominal_unit=V  v_Cds_specify=off  v_Cds_priority=High  v_Cds=0 V  v_Cds_nominal_specify=off  v_Cds_nominal_value=1  v_Cds_nominal_unit=V  v_Cbs_specify=off  v_Cbs_priority=High  v_Cbs=0 V  v_Cbs_nominal_specify=off  v_Cbs_nominal_value=1  v_Cbs_nominal_unit=V  thermal_network_parameterization=ee.enum.thermalNetworkTopology.junctionCase  Rth=[0, 10] K/W  Rth_Cauer=[1, 3, 10] K/W  Rth_Foster=[.08, .14, .22, .16] K/W  thermal_mass_parameterization=ee.enum.thermalNetwork.timeconstant  thermal_mass=[0, 1] J/K  thermal_mass_Cauer=[.1, .3, 1] J/K  thermal_mass_Foster=[.001, .005, .05, .5] J/K  thermal_time_constant=[0, 10] s  thermal_time_constant_Cauer=[1, 3, 10] s  thermal_time_constant_Foster=[7e-05, .0007, .01, .08] s  thermal_mass_initial_temperatures=[25, 25] degC  thermal_mass_initial_temperatures_Cauer=[25, 25, 25] degC  Tvec_initial_Foster=[25, 25, 25, 25] degC  betaref=18 A/V^2  Vfbref=-1.1 V  gamma=3.5 V^(1/2)  phib2ref=1 V  thesatref=0.4 1/V  alpha=0  Vp=5e-2 V  thesrref=0 1/V  m=8  Tref=25 degC  Rsref=2e-3 Ohm  Rdref=0.17 Ohm  Rgref=8.4 Ohm  Rbref=2e-3 Ohm  Cox=1500 pF  Cgso=100 pF  Cgdo=14 pF  Isref=5.2e-13 A  Cj0=480 pF  Tprm=ee.enum.temperatureParameterization.none  etabet=1.3  Stvfb=5e-4 V/K  Stphib=-8.5e-4 V/K  etasat=1.04  etasr=0.65  etar=0.95  etais=3  Tsim=25 degC  Ig_specify=off  Ig_priority=None  Ig=0 A  Ig_nominal_specify=off  Ig_nominal_value=1  Ig_nominal_unit=nA  Ids_specify=off  Ids_priority=None  Ids=0 A  Ids_nominal_specify=off  Ids_nominal_value=1  Ids_nominal_unit=A  Ib_specify=off  Ib_priority=None  Ib=0 A  Ib_nominal_specify=off  Ib_nominal_value=1  Ib_nominal_unit=uA  V_gs_specify=off  V_gs_priority=None  V_gs=0 V  V_gs_nominal_specify=off  V_gs_nominal_value=1  V_gs_nominal_unit=V  V_ds_specify=off  V_ds_priority=None  V_ds=0 V  V_ds_nominal_specify=off  V_ds_nominal_value=1  V_ds_nominal_unit=V  V_bs_specify=off  V_bs_priority=None  V_bs=0 V  V_bs_nominal_specify=off  V_bs_nominal_value=1  V_bs_nominal_unit=V  QGoverCox_specify=off  QGoverCox_priority=None  QGoverCox=0 V  QGoverCox_nominal_specify=off  QGoverCox_nominal_value=1  QGoverCox_nominal_unit=V  QDoverCox_specify=off  QDoverCox_priority=None  QDoverCox=0 V  QDoverCox_nominal_specify=off  QDoverCox_nominal_value=1  QDoverCox_nominal_unit=V  QBoverCox_specify=off  QBoverCox_priority=None  QBoverCox=0 V  QBoverCox_nominal_specify=off  QBoverCox_nominal_value=1  QBoverCox_nominal_unit=V  T0=[25, 25] degC  T0_Cauer=[25, 25, 25] degC
  L 17,71 mH : fl_lib/Electrical/Electrical Elements/Inductor  l=L_ind H  r=r_ind Ohm  g=0 1/Ohm  i_specify=off  i_priority=None  i=0 A  i_nominal_specify=off  i_nominal_value=1  i_nominal_unit=A  v_specify=off  v_priority=None  v=0 V  v_nominal_specify=off  v_nominal_value=1  v_nominal_unit=V  i_L_specify=off  i_L_priority=High  i_L=0 A  i_L_nominal_specify=off  i_L_nominal_value=1  i_L_nominal_unit=A
  Mux medidas : Mux  Inputs=3
  PS-S 1 : nesl_utility/PS-Simulink Converter  PhysicalDomain=network_engine_domain  SubClassName=ps_output  LeftPortType=input  RightPortType=output  PseudoPeriodic=off  Frequencies=[]  VectorFormat=inherit  Unit=V  AffineConversion=off
  PS-S 2 : nesl_utility/PS-Simulink Converter  PhysicalDomain=network_engine_domain  SubClassName=ps_output  LeftPortType=input  RightPortType=output  PseudoPeriodic=off  Frequencies=[]  VectorFormat=inherit  Unit=A  AffineConversion=off
  PS-S 3 : nesl_utility/PS-Simulink Converter  PhysicalDomain=network_engine_domain  SubClassName=ps_output  LeftPortType=input  RightPortType=output  PseudoPeriodic=off  Frequencies=[]  VectorFormat=inherit  Unit=V  AffineConversion=off
  R47 46,6 ohm : fl_lib/Electrical/Electrical Elements/Resistor  R=R_pot Ohm  i_specify=off  i_priority=None  i=0 A  i_nominal_specify=off  i_nominal_value=1  i_nominal_unit=A  v_specify=off  v_priority=None  v=0 V  v_nominal_specify=off  v_nominal_value=1  v_nominal_unit=V
  V no SW : fl_lib/Electrical/Electrical Sensors/Voltage Sensor
  V saida : fl_lib/Electrical/Electrical Sensors/Voltage Sensor
  sensor iL (shunt) : fl_lib/Electrical/Electrical Sensors/Current Sensor
  E : PMIOPort  Side=Left
  GATE : PMIOPort  Port=2  Side=Left
  Vo : PMIOPort  Port=3  Side=Right
  terra de potencia : PMIOPort  Port=4  Side=Right
  medidas : Outport
  wires:
  Mux medidas/1 -> medidas/1
  PS-S 1/1 -> Mux medidas/1
  PS-S 2/1 -> Mux medidas/2
  PS-S 3/1 -> Mux medidas/3
  connections:
  C 470 uF/LConn1 -- E/RConn1 -- C 1 uF (entrada)/LConn1 -- IRF9530/RConn1
  C 470 uF/RConn1 -- C 1 uF (entrada)/RConn1 -- FCH20A20 (roda livre)/LConn1 -- C 4,7 uF/RConn1 -- C 1 uF/RConn1 -- R47 46,6 ohm/RConn1 -- V no SW/RConn2 -- terra de potencia/RConn1 -- V saida/RConn2
  GATE/RConn1 -- IRF9530/LConn1
  FCH20A20 (roda livre)/RConn1 -- IRF9530/RConn2 -- sensor iL (shunt)/LConn1 -- V no SW/LConn1
  sensor iL (shunt)/RConn2 -- L 17,71 mH/LConn1
  C 4,7 uF/LConn1 -- L 17,71 mH/RConn1 -- C 1 uF/LConn1 -- R47 46,6 ohm/LConn1 -- Vo/RConn1 -- V saida/LConn1
  V no SW/RConn1 -- PS-S 1/LConn1
  sensor iL (shunt)/RConn1 -- PS-S 2/LConn1
  V saida/RConn1 -- PS-S 3/LConn1

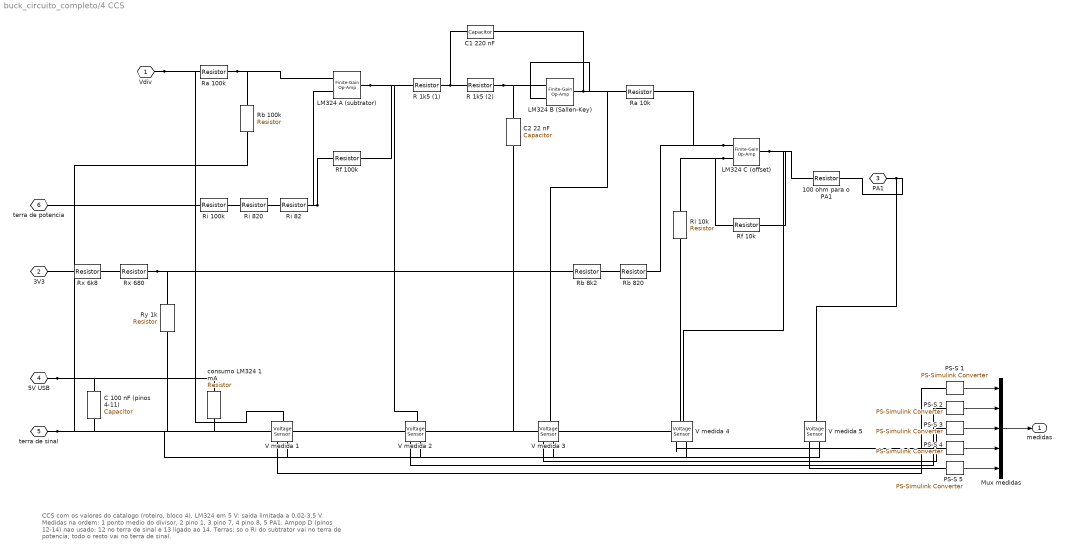
== system buck_circuito_completo/4 CCS ==
  note: CCS com os valores do catalogo (roteiro, bloco 4). LM324 em 5 V: saida limitada a 0,02-3,5 V.
      | Medidas na ordem: 1 ponto medio do divisor, 2 pino 1, 3 pino 7, 4 pino 8, 5 PA1.
      | Ampop D (pinos 12-14) nao usado: 12 no terra de sinal e 13 ligado ao 14.
      | Terras: so o Ri do subtrator vai no terra de potencia; todo o resto vai no terra de sinal.
  100 ohm para o PA1 : fl_lib/Electrical/Electrical Elements/Resistor  R=100 Ohm  i_specify=off  i_priority=None  i=0 A  i_nominal_specify=off  i_nominal_value=1  i_nominal_unit=A  v_specify=off  v_priority=None  v=0 V  v_nominal_specify=off  v_nominal_value=1  v_nominal_unit=V
  C 100 nF (pinos 4-11) : fl_lib/Electrical/Electrical Elements/Capacitor  c=100e-9 F  r=1e-6 Ohm  g=0 1/Ohm  i_specify=off  i_priority=None  i=0 A  i_nominal_specify=off  i_nominal_value=1  i_nominal_unit=A  v_specify=off  v_priority=None  v=0 V  v_nominal_specify=off  v_nominal_value=1  v_nominal_unit=V  vc_specify=off  vc_priority=High  vc=0 V  vc_nominal_specify=off  vc_nominal_value=1  vc_nominal_unit=V
  C1 220 nF : fl_lib/Electrical/Electrical Elements/Capacitor  c=220e-9 F  r=1e-6 Ohm  g=0 1/Ohm  i_specify=off  i_priority=None  i=0 A  i_nominal_specify=off  i_nominal_value=1  i_nominal_unit=A  v_specify=off  v_priority=None  v=0 V  v_nominal_specify=off  v_nominal_value=1  v_nominal_unit=V  vc_specify=off  vc_priority=High  vc=0 V  vc_nominal_specify=off  vc_nominal_value=1  vc_nominal_unit=V
  C2 22 nF : fl_lib/Electrical/Electrical Elements/Capacitor  c=22e-9 F  r=1e-6 Ohm  g=0 1/Ohm  i_specify=off  i_priority=None  i=0 A  i_nominal_specify=off  i_nominal_value=1  i_nominal_unit=A  v_specify=off  v_priority=None  v=0 V  v_nominal_specify=off  v_nominal_value=1  v_nominal_unit=V  vc_specify=off  vc_priority=High  vc=0 V  vc_nominal_specify=off  vc_nominal_value=1  vc_nominal_unit=V
  LM324 A (subtrator) : ee_lib/Integrated Circuits/Finite-Gain Op-Amp  A=1e5  Rin=1e9 Ohm  Rout=100 Ohm  Vmin=0.02 V  Vmax=3.5 V  noise_mode=ee.enum.mode.disabled  v_noise=30e-9 V/Hz^(1/2)  noise_prm=ee.enum.ic.noiseParameterization.same  i_noise=0.5e-12 A/Hz^(1/2)  ip_noise=0.5e-12 A/Hz^(1/2)  in_noise=0.5e-12 A/Hz^(1/2)  sample_time=1e-3 s  repeatability=ee.enum.ic.repeatability.notRepeatable  auto_seed_v=3499211588  auto_seed_ip=3890346746  auto_seed_in=545404223  user_seed_v=0  user_seed_ip=0  user_seed_in=0
  LM324 B (Sallen-Key) : ee_lib/Integrated Circuits/Finite-Gain Op-Amp  A=1e5  Rin=1e9 Ohm  Rout=100 Ohm  Vmin=0.02 V  Vmax=3.5 V  noise_mode=ee.enum.mode.disabled  v_noise=30e-9 V/Hz^(1/2)  noise_prm=ee.enum.ic.noiseParameterization.same  i_noise=0.5e-12 A/Hz^(1/2)  ip_noise=0.5e-12 A/Hz^(1/2)  in_noise=0.5e-12 A/Hz^(1/2)  sample_time=1e-3 s  repeatability=ee.enum.ic.repeatability.notRepeatable  auto_seed_v=3922919431  auto_seed_ip=2715962282  auto_seed_in=418932850  user_seed_v=0  user_seed_ip=0  user_seed_in=0
  LM324 C (offset) : ee_lib/Integrated Circuits/Finite-Gain Op-Amp  A=1e5  Rin=1e9 Ohm  Rout=100 Ohm  Vmin=0.02 V  Vmax=3.5 V  noise_mode=ee.enum.mode.disabled  v_noise=30e-9 V/Hz^(1/2)  noise_prm=ee.enum.ic.noiseParameterization.same  i_noise=0.5e-12 A/Hz^(1/2)  ip_noise=0.5e-12 A/Hz^(1/2)  in_noise=0.5e-12 A/Hz^(1/2)  sample_time=1e-3 s  repeatability=ee.enum.ic.repeatability.notRepeatable  auto_seed_v=1196140742  auto_seed_ip=2348838240  auto_seed_in=4112460543  user_seed_v=0  user_seed_ip=0  user_seed_in=0
  Mux medidas : Mux  Inputs=5
  PS-S {1..5} (5 alike) : nesl_utility/PS-Simulink Converter  PhysicalDomain=network_engine_domain  SubClassName=ps_output  LeftPortType=input  RightPortType=output  PseudoPeriodic=off  Frequencies=[]  VectorFormat=inherit  Unit=V  AffineConversion=off
  R 1k5 (1) : fl_lib/Electrical/Electrical Elements/Resistor  R=1.5e3 Ohm  i_specify=off  i_priority=None  i=0 A  i_nominal_specify=off  i_nominal_value=1  i_nominal_unit=A  v_specify=off  v_priority=None  v=0 V  v_nominal_specify=off  v_nominal_value=1  v_nominal_unit=V
  R 1k5 (2) : fl_lib/Electrical/Electrical Elements/Resistor  R=1.5e3 Ohm  i_specify=off  i_priority=None  i=0 A  i_nominal_specify=off  i_nominal_value=1  i_nominal_unit=A  v_specify=off  v_priority=None  v=0 V  v_nominal_specify=off  v_nominal_value=1  v_nominal_unit=V
  Ra 100k : fl_lib/Electrical/Electrical Elements/Resistor  R=100e3 Ohm  i_specify=off  i_priority=None  i=0 A  i_nominal_specify=off  i_nominal_value=1  i_nominal_unit=A  v_specify=off  v_priority=None  v=0 V  v_nominal_specify=off  v_nominal_value=1  v_nominal_unit=V
  Ra 10k : fl_lib/Electrical/Electrical Elements/Resistor  R=10e3 Ohm  i_specify=off  i_priority=None  i=0 A  i_nominal_specify=off  i_nominal_value=1  i_nominal_unit=A  v_specify=off  v_priority=None  v=0 V  v_nominal_specify=off  v_nominal_value=1  v_nominal_unit=V
  Rb 100k : fl_lib/Electrical/Electrical Elements/Resistor  R=100e3 Ohm  i_specify=off  i_priority=None  i=0 A  i_nominal_specify=off  i_nominal_value=1  i_nominal_unit=A  v_specify=off  v_priority=None  v=0 V  v_nominal_specify=off  v_nominal_value=1  v_nominal_unit=V
  Rb 820 : fl_lib/Electrical/Electrical Elements/Resistor  R=820 Ohm  i_specify=off  i_priority=None  i=0 A  i_nominal_specify=off  i_nominal_value=1  i_nominal_unit=A  v_specify=off  v_priority=None  v=0 V  v_nominal_specify=off  v_nominal_value=1  v_nominal_unit=V
  Rb 8k2 : fl_lib/Electrical/Electrical Elements/Resistor  R=8.2e3 Ohm  i_specify=off  i_priority=None  i=0 A  i_nominal_specify=off  i_nominal_value=1  i_nominal_unit=A  v_specify=off  v_priority=None  v=0 V  v_nominal_specify=off  v_nominal_value=1  v_nominal_unit=V
  Rf 100k : fl_lib/Electrical/Electrical Elements/Resistor  R=100e3 Ohm  i_specify=off  i_priority=None  i=0 A  i_nominal_specify=off  i_nominal_value=1  i_nominal_unit=A  v_specify=off  v_priority=None  v=0 V  v_nominal_specify=off  v_nominal_value=1  v_nominal_unit=V
  Rf 10k : fl_lib/Electrical/Electrical Elements/Resistor  R=10e3 Ohm  i_specify=off  i_priority=None  i=0 A  i_nominal_specify=off  i_nominal_value=1  i_nominal_unit=A  v_specify=off  v_priority=None  v=0 V  v_nominal_specify=off  v_nominal_value=1  v_nominal_unit=V
  Ri 100k : fl_lib/Electrical/Electrical Elements/Resistor  R=100e3 Ohm  i_specify=off  i_priority=None  i=0 A  i_nominal_specify=off  i_nominal_value=1  i_nominal_unit=A  v_specify=off  v_priority=None  v=0 V  v_nominal_specify=off  v_nominal_value=1  v_nominal_unit=V
  Ri 10k : fl_lib/Electrical/Electrical Elements/Resistor  R=10e3 Ohm  i_specify=off  i_priority=None  i=0 A  i_nominal_specify=off  i_nominal_value=1  i_nominal_unit=A  v_specify=off  v_priority=None  v=0 V  v_nominal_specify=off  v_nominal_value=1  v_nominal_unit=V
  Ri 82 : fl_lib/Electrical/Electrical Elements/Resistor  R=82 Ohm  i_specify=off  i_priority=None  i=0 A  i_nominal_specify=off  i_nominal_value=1  i_nominal_unit=A  v_specify=off  v_priority=None  v=0 V  v_nominal_specify=off  v_nominal_value=1  v_nominal_unit=V
  Ri 820 : fl_lib/Electrical/Electrical Elements/Resistor  R=820 Ohm  i_specify=off  i_priority=None  i=0 A  i_nominal_specify=off  i_nominal_value=1  i_nominal_unit=A  v_specify=off  v_priority=None  v=0 V  v_nominal_specify=off  v_nominal_value=1  v_nominal_unit=V
  Rx 680 : fl_lib/Electrical/Electrical Elements/Resistor  R=680 Ohm  i_specify=off  i_priority=None  i=0 A  i_nominal_specify=off  i_nominal_value=1  i_nominal_unit=A  v_specify=off  v_priority=None  v=0 V  v_nominal_specify=off  v_nominal_value=1  v_nominal_unit=V
  Rx 6k8 : fl_lib/Electrical/Electrical Elements/Resistor  R=6.8e3 Ohm  i_specify=off  i_priority=None  i=0 A  i_nominal_specify=off  i_nominal_value=1  i_nominal_unit=A  v_specify=off  v_priority=None  v=0 V  v_nominal_specify=off  v_nominal_value=1  v_nominal_unit=V
  Ry 1k : fl_lib/Electrical/Electrical Elements/Resistor  R=1e3 Ohm  i_specify=off  i_priority=None  i=0 A  i_nominal_specify=off  i_nominal_value=1  i_nominal_unit=A  v_specify=off  v_priority=None  v=0 V  v_nominal_specify=off  v_nominal_value=1  v_nominal_unit=V
  V medida {1..5} (5 alike) : fl_lib/Electrical/Electrical Sensors/Voltage Sensor
  consumo LM324 1 mA : fl_lib/Electrical/Electrical Elements/Resistor  R=5e3 Ohm  i_specify=off  i_priority=None  i=0 A  i_nominal_specify=off  i_nominal_value=1  i_nominal_unit=A  v_specify=off  v_priority=None  v=0 V  v_nominal_specify=off  v_nominal_value=1  v_nominal_unit=V
  Vdiv : PMIOPort  Side=Left
  3V3 : PMIOPort  Port=2  Side=Left
  PA1 : PMIOPort  Port=3  Side=Right
  5V USB : PMIOPort  Port=4  Side=Left
  terra de sinal : PMIOPort  Port=5  Side=Left
  terra de potencia : PMIOPort  Port=6  Side=Left
  medidas : Outport
  wires:
  Mux medidas/1 -> medidas/1
  PS-S 1/1 -> Mux medidas/1
  PS-S 2/1 -> Mux medidas/2
  PS-S 3/1 -> Mux medidas/3
  PS-S 4/1 -> Mux medidas/4
  PS-S 5/1 -> Mux medidas/5
  connections:
  C 100 nF (pinos 4-11)/LConn1 -- 5V USB/RConn1 -- consumo LM324 1 mA/LConn1
  C 100 nF (pinos 4-11)/RConn1 -- consumo LM324 1 mA/RConn1 -- Rb 100k/RConn1 -- C2 22 nF/RConn1 -- Ry 1k/RConn1 -- Ri 10k/RConn1 -- V medida 1/RConn2 -- V medida 2/RConn2 -- V medida 3/RConn2 -- V medida 4/RConn2 -- terra de sinal/RConn1 -- V medida 5/RConn2
  Ra 100k/LConn1 -- Vdiv/RConn1 -- V medida 1/LConn1
  LM324 A (subtrator)/LConn1 -- Ra 100k/RConn1 -- Rb 100k/LConn1
  terra de potencia/RConn1 -- Ri 100k/LConn1
  Ri 100k/RConn1 -- Ri 820/LConn1
  Ri 820/RConn1 -- Ri 82/LConn1
  LM324 A (subtrator)/LConn2 -- Ri 82/RConn1 -- Rf 100k/LConn1
  Rf 100k/RConn1 -- R 1k5 (1)/LConn1 -- LM324 A (subtrator)/RConn1 -- V medida 2/LConn1
  R 1k5 (2)/LConn1 -- R 1k5 (1)/RConn1 -- C1 220 nF/LConn1
  LM324 B (Sallen-Key)/LConn1 -- R 1k5 (2)/RConn1 -- C2 22 nF/LConn1
  LM324 B (Sallen-Key)/LConn2 -- LM324 B (Sallen-Key)/RConn1 -- C1 220 nF/RConn1 -- Ra 10k/LConn1 -- V medida 3/LConn1
  LM324 C (offset)/LConn1 -- Ra 10k/RConn1 -- Rb 820/RConn1
  3V3/RConn1 -- Rx 6k8/LConn1
  Rx 6k8/RConn1 -- Rx 680/LConn1
  Ry 1k/LConn1 -- Rx 680/RConn1 -- Rb 8k2/LConn1
  Rb 8k2/RConn1 -- Rb 820/LConn1
  Ri 10k/LConn1 -- LM324 C (offset)/LConn2 -- Rf 10k/LConn1
  Rf 10k/RConn1 -- 100 ohm para o PA1/LConn1 -- LM324 C (offset)/RConn1 -- V medida 4/LConn1
  PA1/RConn1 -- 100 ohm para o PA1/RConn1 -- V medida 5/LConn1
  V medida 1/RConn1 -- PS-S 1/LConn1
  V medida 2/RConn1 -- PS-S 2/LConn1
  V medida 3/RConn1 -- PS-S 3/LConn1
  V medida 4/RConn1 -- PS-S 4/LConn1
  V medida 5/RConn1 -- PS-S 5/LConn1

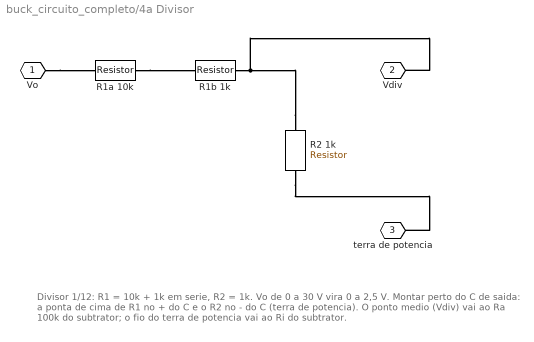
== system buck_circuito_completo/4a Divisor ==
  note: Divisor 1/12: R1 = 10k + 1k em serie, R2 = 1k. Vo de 0 a 30 V vira 0 a 2,5 V.
      | Montar perto do C de saida: a ponta de cima de R1 no + do C e o R2 no - do C (terra de potencia).
      | O ponto medio (Vdiv) vai ao Ra 100k do subtrator; o fio do terra de potencia vai ao Ri do subtrator.
  R1a 10k : fl_lib/Electrical/Electrical Elements/Resistor  R=10e3 Ohm  i_specify=off  i_priority=None  i=0 A  i_nominal_specify=off  i_nominal_value=1  i_nominal_unit=A  v_specify=off  v_priority=None  v=0 V  v_nominal_specify=off  v_nominal_value=1  v_nominal_unit=V
  R1b 1k : fl_lib/Electrical/Electrical Elements/Resistor  R=1e3 Ohm  i_specify=off  i_priority=None  i=0 A  i_nominal_specify=off  i_nominal_value=1  i_nominal_unit=A  v_specify=off  v_priority=None  v=0 V  v_nominal_specify=off  v_nominal_value=1  v_nominal_unit=V
  R2 1k : fl_lib/Electrical/Electrical Elements/Resistor  R=1e3 Ohm  i_specify=off  i_priority=None  i=0 A  i_nominal_specify=off  i_nominal_value=1  i_nominal_unit=A  v_specify=off  v_priority=None  v=0 V  v_nominal_specify=off  v_nominal_value=1  v_nominal_unit=V
  Vo : PMIOPort  Side=Left
  Vdiv : PMIOPort  Port=2  Side=Right
  terra de potencia : PMIOPort  Port=3  Side=Right
  connections:
  Vo/RConn1 -- R1a 10k/LConn1
  R1a 10k/RConn1 -- R1b 1k/LConn1
  R2 1k/LConn1 -- R1b 1k/RConn1 -- Vdiv/RConn1
  R2 1k/RConn1 -- terra de potencia/RConn1
